simulink model "InductionHeating_bb_4"  (R2026b)
settings: Solver=FixedStepDiscrete  StopTime=0.008
PostLoadFcn:
  | Ts = 1e-6;Ts_fpga=10e-9;   R=3; Capa=300e-9;L=100e-6;Pejo_factor=1;
InitFcn:
  | Ts = 1e-6;Ts_fpga=10e-9;   R=3; Capa=300e-9;L=100e-6;Pejo_factor=1;
undefined symbols (not defined in the file or in its folder): DiscIntNeverNeededParam, ee_sli_rtmsupport, gcbh, isSetWhenUndefinedState, MATESOCwDio
libraries: fl_lib x67, nesl_utility x40, hdlsllib x32, simulink x15, eeGeneralControl x9, ee_lib x3
(part 7 of 7)

== system InductionHeating_bb_4/soc16/RLCsw8/mmul8_8 ==
  In1 : Inport
  In2 : Inport  Port=2
  Demux2 : Demux  Outputs=8
  Demux3 : Demux  Outputs=8
  Mux2 : Mux  Inputs=8
  mult{12,15,18..19,21..22,25..26} (8 alike) : Product
  Out1 : Outport
  wires:
  Demux3/3 -> mult18/2
  Demux3/4 -> mult19/2
  mult18/1 -> Mux2/3
  mult21/1 -> Mux2/5
  Demux3/7 -> mult25/2
  mult12/1 -> Mux2/1
  In2/1 -> Demux3/1
  Demux3/1 -> mult12/2
  Demux2/2 -> mult15/1
  Demux2/1 -> mult12/1
  Demux2/8 -> mult26/1
  Demux3/2 -> mult15/2
  Demux2/3 -> mult18/1
  mult22/1 -> Mux2/6
  mult15/1 -> Mux2/2
  mult25/1 -> Mux2/7
  mult19/1 -> Mux2/4
  mult26/1 -> Mux2/8
  Demux2/6 -> mult22/1
  Demux3/5 -> mult21/2
  Demux2/4 -> mult19/1
  Demux2/7 -> mult25/1
  Demux2/5 -> mult21/1
  Demux3/8 -> mult26/2
  Demux3/6 -> mult22/2
  In1/1 -> Demux2/1
  Mux2/1 -> Out1/1

== system InductionHeating_bb_4/soc16/RLCsw8/mmul8_9 ==
  In1 : Inport
  In2 : Inport  Port=2
  Demux2 : Demux  Outputs=8
  Demux3 : Demux  Outputs=8
  Mux2 : Mux  Inputs=8
  mult{12,15,18..19,21..22,25..26} (8 alike) : Product
  Out1 : Outport
  wires:
  Mux2/1 -> Out1/1
  In1/1 -> Demux2/1
  Demux3/6 -> mult22/2
  Demux3/8 -> mult26/2
  Demux2/5 -> mult21/1
  Demux2/7 -> mult25/1
  Demux2/4 -> mult19/1
  Demux3/5 -> mult21/2
  Demux2/6 -> mult22/1
  mult26/1 -> Mux2/8
  mult19/1 -> Mux2/4
  mult25/1 -> Mux2/7
  mult15/1 -> Mux2/2
  mult22/1 -> Mux2/6
  Demux2/3 -> mult18/1
  Demux3/2 -> mult15/2
  Demux2/8 -> mult26/1
  Demux2/1 -> mult12/1
  Demux2/2 -> mult15/1
  Demux3/1 -> mult12/2
  In2/1 -> Demux3/1
  mult12/1 -> Mux2/1
  Demux3/7 -> mult25/2
  mult21/1 -> Mux2/5
  mult18/1 -> Mux2/3
  Demux3/4 -> mult19/2
  Demux3/3 -> mult18/2

== system InductionHeating_bb_4/soc16/RLCsw8/no inverse ==
  typ : Inport
  R_Rx_Lx_Cx : Inport  Port=2
  is_sw : Inport  Port=3
  Bus Creator : BusCreator  Inputs=2
  Constant1 : Constant  Value=[1 1 1 1 1 1 1 1]*(-Ts)  OutDataTypeStr=single  SampleTime=Ts
  Constant2 : Constant  Value=0  OutDataTypeStr=single  SampleTime=Ts
  Constant3 : Constant  Value=[1 1 1 1 1 1 1 1]*(-Ts)  OutDataTypeStr=single  SampleTime=Ts
  Constant4 : Constant  Value=[1 1 1 1 1 1 1 1]*(Ts/2)  OutDataTypeStr=single  SampleTime=Ts
  Demux1 : Demux  Outputs=3
  Switch : Switch  Criteria=u2 ~= 0  SaturateOnIntegerOverflow=off  InputSameDT=off
  Switch2 : Switch  Criteria=u2 ~= 0  SaturateOnIntegerOverflow=off  InputSameDT=off
  mmul8_1 : Subsystem
      mask Display: disp('X8')
  mmul8_2 : Subsystem
      mask Display: disp('X8')
  mmul8_3 : Subsystem
      mask Display: disp('X8')
  mmul8_4 : Subsystem
      mask Display: disp('X8')
  mmul8_5 : Subsystem
      mask Display: disp('X8')
  AhB : Outport
  wires:
  Demux1/3 -> mmul8_2/2(In2), mmul8_1/2(In2), mmul8_5/1(In1)  "1/C or 1/L"
  R_Rx_Lx_Cx/1 -> Demux1/1
  typ/1 -> Switch/2
  Switch/1 -> Bus Creator/1  "Ah"
  Bus Creator/1 -> AhB/1
  Demux1/2 -> mmul8_2/1(In1)  "1/R"
  mmul8_1/1(Out1) -> mmul8_3/1(In1)  "R/L"
  mmul8_4/1(Out1) -> Switch/3  "Ah (RC)"
  mmul8_5/1(Out1) -> Bus Creator/2  "Bh/2"
  is_sw/1 -> Switch2/2
  Constant2/1 -> Switch2/1  "a0"
  Demux1/1 -> mmul8_1/1(In1)  "r_sig"
  mmul8_3/1(Out1) -> Switch2/3  "Ah (RL)"
  Switch2/1 -> Switch/1  "Ah"
  Constant1/1 -> mmul8_3/2(In2)  "-Ts"
  mmul8_2/1(Out1) -> mmul8_4/1(In1)  "R/L"
  Constant3/1 -> mmul8_4/2(In2)  "-Ts"
  Constant4/1 -> mmul8_5/2(In2)  "-Ts"

== system InductionHeating_bb_4/soc16/RLCsw8/recip8_1 ==
  In1 : Inport
  Demux2 : Demux  Outputs=8
  Mux2 : Mux  Inputs=8
  mult25_recip{1..8} (8 alike) : Math  Operator=reciprocal
  Out1 : Outport
  wires:
  Mux2/1 -> Out1/1
  In1/1 -> Demux2/1
  Demux2/1 -> mult25_recip1/1
  Demux2/2 -> mult25_recip2/1
  Demux2/3 -> mult25_recip3/1
  Demux2/4 -> mult25_recip4/1
  Demux2/5 -> mult25_recip5/1
  Demux2/6 -> mult25_recip6/1
  Demux2/7 -> mult25_recip7/1
  Demux2/8 -> mult25_recip8/1
  mult25_recip1/1 -> Mux2/1
  mult25_recip2/1 -> Mux2/2
  mult25_recip3/1 -> Mux2/3
  mult25_recip4/1 -> Mux2/4
  mult25_recip5/1 -> Mux2/5
  mult25_recip6/1 -> Mux2/6
  mult25_recip7/1 -> Mux2/7
  mult25_recip8/1 -> Mux2/8

== system InductionHeating_bb_4/soc16/RLCsw8/recip8_2 ==
  In1 : Inport
  Demux2 : Demux  Outputs=8
  Mux2 : Mux  Inputs=8
  mult25_recip{1..8} (8 alike) : Math  Operator=reciprocal
  Out1 : Outport
  wires:
  mult25_recip8/1 -> Mux2/8
  mult25_recip7/1 -> Mux2/7
  mult25_recip6/1 -> Mux2/6
  mult25_recip5/1 -> Mux2/5
  mult25_recip4/1 -> Mux2/4
  mult25_recip3/1 -> Mux2/3
  mult25_recip2/1 -> Mux2/2
  mult25_recip1/1 -> Mux2/1
  Demux2/8 -> mult25_recip8/1
  Demux2/7 -> mult25_recip7/1
  Demux2/6 -> mult25_recip6/1
  Demux2/5 -> mult25_recip5/1
  Demux2/4 -> mult25_recip4/1
  Demux2/3 -> mult25_recip3/1
  Demux2/2 -> mult25_recip2/1
  Demux2/1 -> mult25_recip1/1
  In1/1 -> Demux2/1
  Mux2/1 -> Out1/1

== system InductionHeating_bb_4/soc16/RLCsw8/recip8_3 ==
  In1 : Inport
  Demux2 : Demux  Outputs=8
  Mux2 : Mux  Inputs=8
  mult25_recip{1..8} (8 alike) : Math  Operator=reciprocal
  Out1 : Outport
  wires:
  Mux2/1 -> Out1/1
  In1/1 -> Demux2/1
  Demux2/1 -> mult25_recip1/1
  Demux2/2 -> mult25_recip2/1
  Demux2/3 -> mult25_recip3/1
  Demux2/4 -> mult25_recip4/1
  Demux2/5 -> mult25_recip5/1
  Demux2/6 -> mult25_recip6/1
  Demux2/7 -> mult25_recip7/1
  Demux2/8 -> mult25_recip8/1
  mult25_recip1/1 -> Mux2/1
  mult25_recip2/1 -> Mux2/2
  mult25_recip3/1 -> Mux2/3
  mult25_recip4/1 -> Mux2/4
  mult25_recip5/1 -> Mux2/5
  mult25_recip6/1 -> Mux2/6
  mult25_recip7/1 -> Mux2/7
  mult25_recip8/1 -> Mux2/8

== system InductionHeating_bb_4/soc16/RLCsw8/recip8_4 ==
  In1 : Inport
  Demux2 : Demux  Outputs=8
  Mux2 : Mux  Inputs=8
  mult25_recip{1..8} (8 alike) : Math  Operator=reciprocal
  Out1 : Outport
  wires:
  Mux2/1 -> Out1/1
  In1/1 -> Demux2/1
  Demux2/1 -> mult25_recip1/1
  Demux2/2 -> mult25_recip2/1
  Demux2/3 -> mult25_recip3/1
  Demux2/4 -> mult25_recip4/1
  Demux2/5 -> mult25_recip5/1
  Demux2/6 -> mult25_recip6/1
  Demux2/7 -> mult25_recip7/1
  Demux2/8 -> mult25_recip8/1
  mult25_recip1/1 -> Mux2/1
  mult25_recip2/1 -> Mux2/2
  mult25_recip3/1 -> Mux2/3
  mult25_recip4/1 -> Mux2/4
  mult25_recip5/1 -> Mux2/5
  mult25_recip6/1 -> Mux2/6
  mult25_recip7/1 -> Mux2/7
  mult25_recip8/1 -> Mux2/8

== system InductionHeating_bb_4/soc16/RLCsw8/state_init ==
  in : Inport
  g_port : Inport  Port=2
  Gain18 : Gain
  Relational Operator1 : RelationalOperator  Operator=~=  OutDataTypeStr=boolean  RndMeth=Simplest  InputSameDT=off
  Switch16 : Switch  Criteria=u2 ~= 0  Threshold=0.5  SaturateOnIntegerOverflow=off  InputSameDT=off
  Unit Delay6 : UnitDelay  SampleTime=-1
  Unit Delay7 : UnitDelay  SampleTime=Ts
  Unit Delay8 : UnitDelay  SampleTime=Ts
  init_in : Constant  Value=0  OutDataTypeStr=single  SampleTime=Ts
  out : Outport
  wires:
  g_port/1 -> Relational Operator1/2, Unit Delay8/1
  Switch16/1 -> out/1
  in/1 -> Unit Delay6/1
  Unit Delay7/1 -> Switch16/1
  Gain18/1 -> Switch16/2
  init_in/1 -> Unit Delay7/1
  Unit Delay6/1 -> Switch16/3
  Relational Operator1/1 -> Gain18/1
  Unit Delay8/1 -> Relational Operator1/1

== system InductionHeating_bb_4/MATEwDiode/MATE 2-level inverter/SW/Dynamic dead zone ==
  up : Inport
  u : Inport  Port=2
  lo : Inport  Port=3
  Diff : Sum  Inputs=+-  InputSameDT=on  OutDataTypeStr=Inherit: Same as first input
  Switch4 : Switch  Criteria=u2 ~= 0  ZeroCross=off  SaturateOnIntegerOverflow=off
  Switch5 : Switch  Criteria=u2 ~= 0  ZeroCross=off  SaturateOnIntegerOverflow=off
  u_GTE_up : RelationalOperator  DisableCoverage=on  OutDataTypeStr=boolean  ZeroCross=off  InputSameDT=off
  u_GT_lo : RelationalOperator  DisableCoverage=on  Operator=>  OutDataTypeStr=boolean  ZeroCross=off  InputSameDT=off
  Out : Outport
  wires:
  lo/1 -> u_GT_lo/2, Switch5/3
  up/1 -> Switch4/1, u_GTE_up/2
  u/1 -> Diff/1, u_GTE_up/1, Switch5/1, u_GT_lo/1
  u_GTE_up/1 -> Switch4/2
  Switch4/1 -> Diff/2
  Switch5/1 -> Switch4/3
  Diff/1 -> Out/1
  u_GT_lo/1 -> Switch5/2

== system InductionHeating_bb_4/MATEwDiode/MATE 2-level inverter/SW/INT ==
  u : Inport
  Initial : Inport  Port=2
  en : Inport  Port=3
  Logical Operator10 : Logic  Operator=NOT  AllPortsSameDT=off  OutDataTypeStr=boolean
  Saturation : Saturate  Commented=through  UpperLimit=inf  LowerLimit=0
  Sum : Sum  Inputs=|-+
  Switch1 : Switch  Criteria=u2 ~= 0  SaturateOnIntegerOverflow=off  InputSameDT=off
  Unit Delay1 : UnitDelay  SampleTime=Ts
  u_p : Outport  VectorParamsAs1DForOutWhenUnconnected=off
  wires:
  u/1 -> Sum/1
  en/1 -> Logical Operator10/1
  Saturation/1 -> u_p/1, Unit Delay1/1
  Switch1/1 -> Sum/2
  Sum/1 -> Saturation/1
  Unit Delay1/1 -> Switch1/3
  Initial/1 -> Switch1/1
  Logical Operator10/1 -> Switch1/2

== system InductionHeating_bb_4/soc16/DynamicMultMAT/multdiv1/mmul8_1 ==
  In1 : Inport
  In2 : Inport  Port=2
  Demux2 : Demux  Outputs=8
  Demux3 : Demux  Outputs=8
  Mux2 : Mux  Inputs=8
  Selector : Selector  InputPortWidth=1  IndexOptions=Index vector (dialog)  Indices=[1 1 1 1 1 1 1 1]  OutputSizes=1  RuntimeRangeChecks=off
  mult{12,15,18..19,21..22,25..26} (8 alike) : Product
  Out1 : Outport
  wires:
  Selector/1 -> Demux2/1
  Mux2/1 -> Out1/1
  In1/1 -> Selector/1
  Demux3/6 -> mult22/2
  Demux3/8 -> mult26/2
  Demux2/5 -> mult21/1
  Demux2/7 -> mult25/1
  Demux2/4 -> mult19/1
  Demux3/5 -> mult21/2
  Demux2/6 -> mult22/1
  mult26/1 -> Mux2/8
  mult19/1 -> Mux2/4
  mult25/1 -> Mux2/7
  mult15/1 -> Mux2/2
  mult22/1 -> Mux2/6
  Demux2/3 -> mult18/1
  Demux3/2 -> mult15/2
  Demux2/8 -> mult26/1
  Demux2/1 -> mult12/1
  Demux2/2 -> mult15/1
  Demux3/1 -> mult12/2
  In2/1 -> Demux3/1
  mult12/1 -> Mux2/1
  Demux3/7 -> mult25/2
  mult21/1 -> Mux2/5
  mult18/1 -> Mux2/3
  Demux3/4 -> mult19/2
  Demux3/3 -> mult18/2

== system InductionHeating_bb_4/soc16/DynamicMultMAT/multdiv1/mmul8_11 ==
  In1 : Inport
  In2 : Inport  Port=2
  Demux2 : Demux  Outputs=8
  Demux3 : Demux  Outputs=8
  Mux2 : Mux  Inputs=8
  Selector : Selector  InputPortWidth=1  IndexOptions=Index vector (dialog)  Indices=[1 1 1 1 1 1 1 1]  OutputSizes=1  RuntimeRangeChecks=off
  mult{12,15,18..19,21..22,25..26} (8 alike) : Product
  Out1 : Outport
  wires:
  Demux3/3 -> mult18/2
  Demux3/4 -> mult19/2
  mult18/1 -> Mux2/3
  mult21/1 -> Mux2/5
  Demux3/7 -> mult25/2
  mult12/1 -> Mux2/1
  In2/1 -> Demux3/1
  Demux3/1 -> mult12/2
  Demux2/2 -> mult15/1
  Demux2/1 -> mult12/1
  Demux2/8 -> mult26/1
  Demux3/2 -> mult15/2
  Demux2/3 -> mult18/1
  mult22/1 -> Mux2/6
  mult15/1 -> Mux2/2
  mult25/1 -> Mux2/7
  mult19/1 -> Mux2/4
  mult26/1 -> Mux2/8
  Demux2/6 -> mult22/1
  Demux3/5 -> mult21/2
  Demux2/4 -> mult19/1
  Demux2/7 -> mult25/1
  Demux2/5 -> mult21/1
  Demux3/8 -> mult26/2
  Demux3/6 -> mult22/2
  In1/1 -> Selector/1
  Mux2/1 -> Out1/1
  Selector/1 -> Demux2/1

== system InductionHeating_bb_4/soc16/MATE 2-level inverter SWFHIZ (3p)/SW/Dynamic dread zone1 ==
  up : Inport
  u_port : Inport  Port=2
  lo : Inport  Port=3
  Diff : Sum  Inputs=+-  InputSameDT=on  OutDataTypeStr=Inherit: Same as first input
  Switch4 : Switch  Criteria=u2 ~= 0  ZeroCross=off  SaturateOnIntegerOverflow=off
  Switch5 : Switch  Criteria=u2 ~= 0  ZeroCross=off  SaturateOnIntegerOverflow=off
  u_GTE_up : RelationalOperator  DisableCoverage=on  OutDataTypeStr=boolean  ZeroCross=off  InputSameDT=off
  u_GT_lo : RelationalOperator  DisableCoverage=on  Operator=>  OutDataTypeStr=boolean  ZeroCross=off  InputSameDT=off
  Out : Outport
  wires:
  u_GT_lo/1 -> Switch5/2
  Diff/1 -> Out/1
  Switch5/1 -> Switch4/3
  Switch4/1 -> Diff/2
  u_GTE_up/1 -> Switch4/2
  u_port/1 -> u_GT_lo/1, Switch5/1, u_GTE_up/1, Diff/1
  up/1 -> u_GTE_up/2, Switch4/1
  lo/1 -> Switch5/3, u_GT_lo/2

== system InductionHeating_bb_4/soc16/MATE 2-level inverter SWFHIZ (3p)/SW/INT ==
  u_port : Inport
  Initial : Inport  Port=2
  en : Inport  Port=3
  Saturation : Saturate  Commented=through  UpperLimit=inf  LowerLimit=0
  Sum : Sum  Inputs=|-+
  Switch1 : Switch  Criteria=u2 ~= 0  SaturateOnIntegerOverflow=off  InputSameDT=off
  Unit Delay1 : UnitDelay  SampleTime=Ts
  u_p : Outport  VectorParamsAs1DForOutWhenUnconnected=off
  wires:
  en/1 -> Switch1/2
  Sum/1 -> Saturation/1
  Switch1/1 -> Sum/2
  Saturation/1 -> Unit Delay1/1, u_p/1
  u_port/1 -> Sum/1
  Unit Delay1/1 -> Switch1/1
  Initial/1 -> Switch1/3

== system InductionHeating_bb_4/soc16/MATE 2-level inverter SWFHIZ (3p)/SW/Set-Reset Flip-Flop ==
  Set : Inport
  Reset : Inport  Port=2
  Continuous : Subsystem  VariantControl=Continuous
  Discrete : Subsystem  VariantControl=Discrete
  q_port : Outport  VectorParamsAs1DForOutWhenUnconnected=off
  !Q : Outport  Port=2  VectorParamsAs1DForOutWhenUnconnected=off

== system InductionHeating_bb_4/soc16/MATE 2-level inverter SWFHIZ (3p)/SW1/Dynamic dead zone ==
  up : Inport
  u : Inport  Port=2
  lo : Inport  Port=3
  Diff : Sum  Inputs=+-  InputSameDT=on  OutDataTypeStr=Inherit: Same as first input
  Switch4 : Switch  Criteria=u2 ~= 0  ZeroCross=off  SaturateOnIntegerOverflow=off
  Switch5 : Switch  Criteria=u2 ~= 0  ZeroCross=off  SaturateOnIntegerOverflow=off
  u_GTE_up : RelationalOperator  DisableCoverage=on  OutDataTypeStr=boolean  ZeroCross=off  InputSameDT=off
  u_GT_lo : RelationalOperator  DisableCoverage=on  Operator=>  OutDataTypeStr=boolean  ZeroCross=off  InputSameDT=off
  Out : Outport
  wires:
  lo/1 -> u_GT_lo/2, Switch5/3
  up/1 -> Switch4/1, u_GTE_up/2
  u/1 -> Diff/1, u_GTE_up/1, Switch5/1, u_GT_lo/1
  u_GTE_up/1 -> Switch4/2
  Switch4/1 -> Diff/2
  Switch5/1 -> Switch4/3
  Diff/1 -> Out/1
  u_GT_lo/1 -> Switch5/2

== system InductionHeating_bb_4/soc16/MATE 2-level inverter SWFHIZ (3p)/SW1/INT ==
  u : Inport
  Initial : Inport  Port=2
  en : Inport  Port=3
  Logical Operator10 : Logic  Operator=NOT  AllPortsSameDT=off  OutDataTypeStr=boolean
  Saturation : Saturate  Commented=through  UpperLimit=inf  LowerLimit=0
  Sum : Sum  Inputs=|-+
  Switch1 : Switch  Criteria=u2 ~= 0  SaturateOnIntegerOverflow=off  InputSameDT=off
  Unit Delay1 : UnitDelay  SampleTime=Ts
  u_p : Outport  VectorParamsAs1DForOutWhenUnconnected=off
  wires:
  u/1 -> Sum/1
  en/1 -> Logical Operator10/1
  Saturation/1 -> u_p/1, Unit Delay1/1
  Switch1/1 -> Sum/2
  Sum/1 -> Saturation/1
  Unit Delay1/1 -> Switch1/3
  Initial/1 -> Switch1/1
  Logical Operator10/1 -> Switch1/2

== system InductionHeating_bb_4/soc16/RLCsw8/Diode2/Pejovic L-C-switch component ==
  gate : Inport
  Vf : Inport  Port=2
  Add : Sum  Inputs=+-
  Add1 : Sum  Inputs=2
  Add2 : Sum  Inputs=+-
  Add3 : Sum  Inputs=2
  Add4 : Sum  Inputs=+-
  CCS1 : fl_lib/Electrical/Electrical Sources/Controlled Current Source
  Gain1 : Gain  Gain=-1/Rsw
  Gain2 : Gain  Gain=Xcomp
  Gain3 : Gain  Gain=-1
  Gain4 : Gain  Gain=-1
  Gain5 : Gain  Gain=1/Rsw*traprule
  Gain6 : Gain  Gain=traprule
  Gain7 : Gain  Gain=-1/Rsw
  PS-Simulink Converter2 : nesl_utility/PS-Simulink Converter  PhysicalDomain=network_engine_domain  SubClassName=ps_output  LeftPortType=input  RightPortType=output  PseudoPeriodic=off  Frequencies=[]  VectorFormat=inherit  Unit=inherit  AffineConversion=off
  Relational Operator1 : RelationalOperator  Operator=~=  OutDataTypeStr=boolean  RndMeth=Simplest  InputSameDT=off
  Resistor : fl_lib/Electrical/Electrical Elements/Resistor  R=Rsw Ohm  i_specify=off  i_priority=None  i=0 A  i_nominal_specify=off  i_nominal_value=1  i_nominal_unit=A  v_specify=off  v_priority=None  v=0 V  v_nominal_specify=off  v_nominal_value=1  v_nominal_unit=V
  Simulink-PS Converter1 : nesl_utility/Simulink-PS Converter  PhysicalDomain=network_engine_domain  SubClassName=ps_input  LeftPortType=input  RightPortType=output  PseudoPeriodic=off  Frequencies=[]  NoiseDistribution=none  NoiseParameters=[]  Unit=1  AffineConversion=off  FilteringAndDerivatives=provide  SimscapeFilterOrder=1  InputFilterTimeConstant=0.001  UdotUserProvided=0
  Switch : Switch  Criteria=u2 > Threshold  Threshold=0.5  SaturateOnIntegerOverflow=off  InputSameDT=off
  Switch4 : Switch  Criteria=u2 > Threshold  Threshold=0.5  SaturateOnIntegerOverflow=off  InputSameDT=off
  Switch5 : Switch  Criteria=u2 ~= 0  Threshold=0.5  SaturateOnIntegerOverflow=off  InputSameDT=off
  Unit Delay1 : UnitDelay  SampleTime=-1
  Unit Delay2 : UnitDelay  SampleTime=Ts
  Unit Delay6 : UnitDelay  SampleTime=Ts
  VS1 : fl_lib/Electrical/Electrical Sensors/Voltage Sensor
  init_in : Constant
  init_out : Terminator
  +V : PMIOPort  Side=Left
  -V : PMIOPort  Port=2  Side=Right
  v : Outport
  i : Outport  Port=2
  wires:
  Unit Delay2/1 -> Switch5/1
  [Ihist] -> Gain3/1, Switch4/3
  Add/1 -> Gain6/1, Add1/1, Gain4/1
  Switch/1 -> Unit Delay1/1
  [Vsw] -> Gain1/1
  PS-Simulink Converter2/1 -> Add4/1
  [Ihist] -> Add/1
  Gain1/1 -> Add2/1, Add/2
  Unit Delay1/1 -> Switch5/3
  Switch4/1 -> init_out/1
  Gain3/1 -> Switch4/1
  Gain2/1 -> Switch5/2
  Unit Delay6/1 -> Relational Operator1/1
  gate/1 -> Switch4/2, Unit Delay6/1, Relational Operator1/2, Switch/2
  Relational Operator1/1 -> Gain2/1
  init_in/1 -> Unit Delay2/1
  Switch5/1 -> [Ihist]
  Gain4/1 -> i/1
  Add1/1 -> Switch/1
  [Vsw] -> Gain5/1
  Gain5/1 -> Add1/2
  Add2/1 -> Switch/3
  Gain6/1 -> Add2/2
  Vf/1 -> Add4/2, Gain7/1
  [Ihist] -> Add3/1
  Gain7/1 -> Add3/2
  Add3/1 -> Simulink-PS Converter1/1
  Add4/1 -> v/1, [Vsw]
  connections:
  CCS1/RConn2 -- +V/RConn1 -- VS1/LConn1 -- Resistor/LConn1
  CCS1/RConn1 -- Simulink-PS Converter1/RConn1
  PS-Simulink Converter2/LConn1 -- VS1/RConn1
  -V/RConn1 -- VS1/RConn2 -- CCS1/LConn1 -- Resistor/RConn1

== system InductionHeating_bb_4/soc16/RLCsw8/no inverse/mmul8_1 ==
  In1 : Inport
  In2 : Inport  Port=2
  Demux2 : Demux  Outputs=8
  Demux3 : Demux  Outputs=8
  Mux2 : Mux  Inputs=8
  mult{12,15,18..19,21..22,25..26} (8 alike) : Product
  Out1 : Outport
  wires:
  Demux3/3 -> mult18/2
  Demux3/4 -> mult19/2
  mult18/1 -> Mux2/3
  mult21/1 -> Mux2/5
  Demux3/7 -> mult25/2
  mult12/1 -> Mux2/1
  In2/1 -> Demux3/1
  Demux3/1 -> mult12/2
  Demux2/2 -> mult15/1
  Demux2/1 -> mult12/1
  Demux2/8 -> mult26/1
  Demux3/2 -> mult15/2
  Demux2/3 -> mult18/1
  mult22/1 -> Mux2/6
  mult15/1 -> Mux2/2
  mult25/1 -> Mux2/7
  mult19/1 -> Mux2/4
  mult26/1 -> Mux2/8
  Demux2/6 -> mult22/1
  Demux3/5 -> mult21/2
  Demux2/4 -> mult19/1
  Demux2/7 -> mult25/1
  Demux2/5 -> mult21/1
  Demux3/8 -> mult26/2
  Demux3/6 -> mult22/2
  In1/1 -> Demux2/1
  Mux2/1 -> Out1/1

== system InductionHeating_bb_4/soc16/RLCsw8/no inverse/mmul8_2 ==
  In1 : Inport
  In2 : Inport  Port=2
  Demux2 : Demux  Outputs=8
  Demux3 : Demux  Outputs=8
  Mux2 : Mux  Inputs=8
  mult{12,15,18..19,21..22,25..26} (8 alike) : Product
  Out1 : Outport
  wires:
  Mux2/1 -> Out1/1
  In1/1 -> Demux2/1
  Demux3/6 -> mult22/2
  Demux3/8 -> mult26/2
  Demux2/5 -> mult21/1
  Demux2/7 -> mult25/1
  Demux2/4 -> mult19/1
  Demux3/5 -> mult21/2
  Demux2/6 -> mult22/1
  mult26/1 -> Mux2/8
  mult19/1 -> Mux2/4
  mult25/1 -> Mux2/7
  mult15/1 -> Mux2/2
  mult22/1 -> Mux2/6
  Demux2/3 -> mult18/1
  Demux3/2 -> mult15/2
  Demux2/8 -> mult26/1
  Demux2/1 -> mult12/1
  Demux2/2 -> mult15/1
  Demux3/1 -> mult12/2
  In2/1 -> Demux3/1
  mult12/1 -> Mux2/1
  Demux3/7 -> mult25/2
  mult21/1 -> Mux2/5
  mult18/1 -> Mux2/3
  Demux3/4 -> mult19/2
  Demux3/3 -> mult18/2

== system InductionHeating_bb_4/soc16/RLCsw8/no inverse/mmul8_3 ==
  In1 : Inport
  In2 : Inport  Port=2
  Demux2 : Demux  Outputs=8
  Demux3 : Demux  Outputs=8
  Mux2 : Mux  Inputs=8
  mult{12,15,18..19,21..22,25..26} (8 alike) : Product
  Out1 : Outport
  wires:
  Demux3/3 -> mult18/2
  Demux3/4 -> mult19/2
  mult18/1 -> Mux2/3
  mult21/1 -> Mux2/5
  Demux3/7 -> mult25/2
  mult12/1 -> Mux2/1
  In2/1 -> Demux3/1
  Demux3/1 -> mult12/2
  Demux2/2 -> mult15/1
  Demux2/1 -> mult12/1
  Demux2/8 -> mult26/1
  Demux3/2 -> mult15/2
  Demux2/3 -> mult18/1
  mult22/1 -> Mux2/6
  mult15/1 -> Mux2/2
  mult25/1 -> Mux2/7
  mult19/1 -> Mux2/4
  mult26/1 -> Mux2/8
  Demux2/6 -> mult22/1
  Demux3/5 -> mult21/2
  Demux2/4 -> mult19/1
  Demux2/7 -> mult25/1
  Demux2/5 -> mult21/1
  Demux3/8 -> mult26/2
  Demux3/6 -> mult22/2
  In1/1 -> Demux2/1
  Mux2/1 -> Out1/1

== system InductionHeating_bb_4/soc16/RLCsw8/no inverse/mmul8_4 ==
  In1 : Inport
  In2 : Inport  Port=2
  Demux2 : Demux  Outputs=8
  Demux3 : Demux  Outputs=8
  Mux2 : Mux  Inputs=8
  mult{12,15,18..19,21..22,25..26} (8 alike) : Product
  Out1 : Outport
  wires:
  Mux2/1 -> Out1/1
  In1/1 -> Demux2/1
  Demux3/6 -> mult22/2
  Demux3/8 -> mult26/2
  Demux2/5 -> mult21/1
  Demux2/7 -> mult25/1
  Demux2/4 -> mult19/1
  Demux3/5 -> mult21/2
  Demux2/6 -> mult22/1
  mult26/1 -> Mux2/8
  mult19/1 -> Mux2/4
  mult25/1 -> Mux2/7
  mult15/1 -> Mux2/2
  mult22/1 -> Mux2/6
  Demux2/3 -> mult18/1
  Demux3/2 -> mult15/2
  Demux2/8 -> mult26/1
  Demux2/1 -> mult12/1
  Demux2/2 -> mult15/1
  Demux3/1 -> mult12/2
  In2/1 -> Demux3/1
  mult12/1 -> Mux2/1
  Demux3/7 -> mult25/2
  mult21/1 -> Mux2/5
  mult18/1 -> Mux2/3
  Demux3/4 -> mult19/2
  Demux3/3 -> mult18/2

== system InductionHeating_bb_4/soc16/RLCsw8/no inverse/mmul8_5 ==
  In1 : Inport
  In2 : Inport  Port=2
  Demux2 : Demux  Outputs=8
  Demux3 : Demux  Outputs=8
  Mux2 : Mux  Inputs=8
  mult{12,15,18..19,21..22,25..26} (8 alike) : Product
  Out1 : Outport
  wires:
  Mux2/1 -> Out1/1
  In1/1 -> Demux2/1
  Demux3/6 -> mult22/2
  Demux3/8 -> mult26/2
  Demux2/5 -> mult21/1
  Demux2/7 -> mult25/1
  Demux2/4 -> mult19/1
  Demux3/5 -> mult21/2
  Demux2/6 -> mult22/1
  mult26/1 -> Mux2/8
  mult19/1 -> Mux2/4
  mult25/1 -> Mux2/7
  mult15/1 -> Mux2/2
  mult22/1 -> Mux2/6
  Demux2/3 -> mult18/1
  Demux3/2 -> mult15/2
  Demux2/8 -> mult26/1
  Demux2/1 -> mult12/1
  Demux2/2 -> mult15/1
  Demux3/1 -> mult12/2
  In2/1 -> Demux3/1
  mult12/1 -> Mux2/1
  Demux3/7 -> mult25/2
  mult21/1 -> Mux2/5
  mult18/1 -> Mux2/3
  Demux3/4 -> mult19/2
  Demux3/3 -> mult18/2

== system InductionHeating_bb_4/soc16/MATE 2-level inverter SWFHIZ (3p)/SW/Set-Reset Flip-Flop/Continuous ==
  Set : Inport  SampleTime=Ts
  Reset : Inport  Port=2  SampleTime=Ts
  Constant : Constant  Value=isSetWhenUndefinedState  SampleTime=Ts
  Data Type Conversion : DataTypeConversion  OutDataTypeStr=boolean  SaturateOnIntegerOverflow=off  RndMeth=Floor
  Data Type Conversion1 : DataTypeConversion  OutDataTypeStr=boolean  SaturateOnIntegerOverflow=off  RndMeth=Floor
  Logical Operator : Logic  Operator=NOT  AllPortsSameDT=off  OutDataTypeStr=boolean
  Logical Operator1 : Logic  AllPortsSameDT=off  OutDataTypeStr=boolean
  Logical Operator2 : Logic  Operator=OR  AllPortsSameDT=off  OutDataTypeStr=boolean
  Logical Operator3 : Logic  Operator=NOT  AllPortsSameDT=off  OutDataTypeStr=boolean
  Logical Operator4 : Logic  Operator=OR  AllPortsSameDT=off  OutDataTypeStr=boolean
  Logical Operator5 : Logic  AllPortsSameDT=off  OutDataTypeStr=boolean
  Memory : Memory  InitialCondition=Q0
  Switch : Switch  Criteria=u2 ~= 0  Threshold=1  SaturateOnIntegerOverflow=off  InputSameDT=off
  q_port : Outport  VectorParamsAs1DForOutWhenUnconnected=off
  !Q : Outport  Port=2  VectorParamsAs1DForOutWhenUnconnected=off
  wires:
  Data Type Conversion1/1 -> Logical Operator/1
  Data Type Conversion/1 -> Logical Operator2/1, Logical Operator4/1
  Memory/1 -> Logical Operator2/2, Logical Operator5/2
  Logical Operator4/1 -> Switch/1
  Logical Operator2/1 -> Logical Operator1/1
  Constant/1 -> Switch/2
  Logical Operator/1 -> Logical Operator1/2, Logical Operator5/1
  Set/1 -> Data Type Conversion/1
  Logical Operator5/1 -> Logical Operator4/2
  Reset/1 -> Data Type Conversion1/1
  Switch/1 -> Logical Operator3/1, Memory/1, q_port/1
  Logical Operator1/1 -> Switch/3
  Logical Operator3/1 -> !Q/1

== system InductionHeating_bb_4/soc16/MATE 2-level inverter SWFHIZ (3p)/SW/Set-Reset Flip-Flop/Discrete ==
  Set : Inport  SampleTime=Ts
  Reset : Inport  Port=2  SampleTime=Ts
  Constant : Constant  Value=isSetWhenUndefinedState  SampleTime=Ts
  Data Type Conversion : DataTypeConversion  OutDataTypeStr=boolean  SaturateOnIntegerOverflow=off  RndMeth=Floor
  Data Type Conversion1 : DataTypeConversion  OutDataTypeStr=boolean  SaturateOnIntegerOverflow=off  RndMeth=Floor
  Logical Operator : Logic  Operator=NOT  AllPortsSameDT=off  OutDataTypeStr=boolean
  Logical Operator1 : Logic  AllPortsSameDT=off  OutDataTypeStr=boolean
  Logical Operator2 : Logic  Operator=OR  AllPortsSameDT=off  OutDataTypeStr=boolean
  Logical Operator3 : Logic  Operator=NOT  AllPortsSameDT=off  OutDataTypeStr=boolean
  Logical Operator4 : Logic  Operator=OR  AllPortsSameDT=off  OutDataTypeStr=boolean
  Logical Operator5 : Logic  AllPortsSameDT=off  OutDataTypeStr=boolean
  Unit Delay : UnitDelay  InitialCondition=Q0  SampleTime=-1
  q_port : Outport  VectorParamsAs1DForOutWhenUnconnected=off
  !Q : Outport  Port=2  VectorParamsAs1DForOutWhenUnconnected=off
  wires:
  Data Type Conversion1/1 -> Logical Operator/1
  Data Type Conversion/1 -> Logical Operator4/1, Logical Operator2/1
  Unit Delay/1 -> Logical Operator5/2, Logical Operator2/2
  Logical Operator3/1 -> !Q/1
  Logical Operator1/1 -> ?
  Logical Operator4/1 -> q_port/1, Logical Operator3/1, Unit Delay/1
  Reset/1 -> Data Type Conversion1/1
  Logical Operator5/1 -> Logical Operator4/2
  Set/1 -> Data Type Conversion/1
  Logical Operator/1 -> Logical Operator5/1, Logical Operator1/2
  Constant/1 -> ?
  Logical Operator2/1 -> Logical Operator1/1
